simulink model "UkfSensorlessFOC"  (R2026b)
settings: Solver=FixedStepDiscrete  StopTime=experimentCfg.Duration  FixedStep=experimentCfg.Step
PostLoadFcn:
  | addpath(fullfile(fileparts(get_param(bdroot,'FileName')),'..','parameter'),fullfile(fileparts(get_param(bdroot,'FileName')),'..','build_process'));initialize_extension_foc(bdroot,'ukf');
model workspace (MAT data in the model file):
  bridgeCfg.Rs = 0.5
  bridgeCfg.Ld = 0.001
  bridgeCfg.Lq = 0.001
  bridgeCfg.Flux = 0.035
  bridgeCfg.PolePairs = 4
  bridgeCfg.J = 0.0005
  bridgeCfg.B = 0.0001
  bridgeCfg.Id0 = 0
  bridgeCfg.Iq0 = 0
  bridgeCfg.Speed0 = 0
  bridgeCfg.Position0 = 0.1
  bridgeCfg.Ts = 5e-06
  bridgeCfg.Vdc = 48
  bridgeCfg.DiodeVf = 0.7
  bridgeCfg.DiodeRon = 0.01
  bridgeCfg.MechanicalEnabled = 1
  bridgeCfg.CurrentTolerance = 1e-09
  bridgeCfg.VoltageTolerance = 1e-08
  bridgeCfg.MaxCurrent = 200
  bridgeCfg.MaxSpeed = 1000
  bridgeCfg.MaxAngleStep = 0.1
  bridgeCfg.State0 = [0; 0; 0; 0.1]
  bridgeCfg.Vector = [5e-06; 0.5; 0.001; 0.001; 0.035; 4; 0.0005; 0.0001; 48; 0.7; 0.01; 1; 1e-09; 1e-08; 200; 1000; 0.1]
  currentCfg.Ts = 5e-05
  currentCfg.BandwidthHz = 500
  currentCfg.Kpd = 3.14159265359
  currentCfg.Kpq = 3.14159265359
  currentCfg.Kid = 1570.79632679
  currentCfg.Kiq = 1570.79632679
  currentCfg.Kaw = 20000
  experimentCfg.UseTiming = 1
  experimentCfg.Step = 5e-06
  experimentCfg.Duration = 2.2
  extensionCfg.Kind = 'ukf'
  focCfg.Direction = 1
  focCfg.SpeedReference = 80
  focCfg.SpeedInitial = 0
  focCfg.CommandTime = 0.05
  focCfg.LoadTorque = 0.1
  focCfg.LoadTime = 0.9
  focCfg.Enable = 1
  focCfg.Reset = 0
  focCfg.ObserverEnable = 1
  focCfg.VoltageAlignmentEnable = 1
  focCfg.AlignmentVoltageGain = 0.5
  focCfg.FrameCorrectionTolerance = 1e-10
  fwCfg.BusTimes = 0
  fwCfg.BusValues = 48
  handoverCfg.Ts = 5e-05
  handoverCfg.MinOmega = 100
  handoverCfg.MaxSpeedGap = 80
  handoverCfg.MaxPhaseGap = 0.9
  handoverCfg.MaxResidual = 1.5
  handoverCfg.CaptureTime = 0.01
  handoverCfg.BlendTime = 0.1
  handoverCfg.LossTime = 0.001
  handoverCfg.MaxPhaseInnovation = 0.15
  handoverCfg.AllowFlying = 0
  handoverCfg.Samples = [200; 2000; 20]
  handoverCfg.Vector = [5e-05; 100; 80; 0.9; 1.5; 200; 2000; 20; 0.15; 0]
  handoverCfg.State0 = [0; 0; 0; 0; 0; 0; 0; 0; 0]
  inverterCfg.Vdc = 48
  inverterCfg.MinDuty = 0.02
  inverterCfg.PwmTs = 5e-05
  inverterCfg.LinearLimit = 26.6043004043
  motionCfg.SpeedLimit = 120
  motionCfg.AccelerationLimit = 200
  normalizedInverterCfg.Vdc = 1
  normalizedInverterCfg.MinDuty = 0.02
  normalizedInverterCfg.PwmTs = 5e-05
  normalizedInverterCfg.LinearLimit = 0.554256258422
  observerCfg.Model.Ts = 5e-05
  observerCfg.Model.Rs = 0.5
  observerCfg.Model.L = 0.001
  observerCfg.Model.Flux = 0.035
  observerCfg.Model.PolePairs = 4
  observerCfg.InitialOmega = 0
  observerCfg.InitialAngle = 0
  observerCfg.InitialStd = [1; 1; 500; 0.5]
  observerCfg.ProcessNoiseDensity = [2; 2; 2000; 1e-05]
  observerCfg.MeasurementStd = [0.002; 0.002]
  observerCfg.QualificationTime = 0.02
  observerCfg.MinOmega = 30
  observerCfg.MinEmf = 1
  observerCfg.MaxNIS = 25
  observerCfg.MaxThetaStd = 0.12
  observerCfg.MaxOmegaStd = 100
  observerCfg.AngleRateTimeConstant = 0.002
  observerCfg.MaxRateMismatch = 60
  observerCfg.MaxOmega = 2000
  observerCfg.MaxInputCurrent = 100
  observerCfg.MaxInputVoltage = 1000
  observerCfg.InitialVariance = [1; 1; 250000; 0.25]
  observerCfg.ProcessVariance = [0.0001; 0.0001; 0.1; 5e-10]
  observerCfg.MeasurementVariance = [4e-06; 4e-06]
  observerCfg.QualificationSamples = 400
  observerCfg.AngleRateAlpha = 0.0243902439024
  observerCfg.Settings = [5e-05; 0.5; 0.001; 0.035; 0; 0; 1; 1; 250000; 0.25; 0.0001; 0.0001; 0.1; 5e-10; 4e-06; 4e-06; 400; 30; 1; 25; 0.12; 100; 0.0243902439024; 60; 2000; 100; 1000]
  observerCfg.Alpha = 1
  observerCfg.Beta = 2
  observerCfg.Kappa = 0
  observerCfg.StateScales = [1; 1; 100; 1]
  observerCfg.InitialJitter = 1e-12
  observerCfg.MaximumJitter = 1e-08
  observerCfg.MaximumJitterAttempts = 5
  observerCfg.MinimumAngleResultant = 1e-06
  observerCfg.MaximumSigmaAngleDeviation = 1.56979632679
  observerCfg.UnscentedSettings = [5e-05; 0.5; 0.001; 0.035; 0; 0; 1; 1; 250000; 0.25; 0.0001; 0.0001; 0.1; 5e-10; 4e-06; 4e-06; 400; 30; 1; 25; 0.12; 100; 0.0243902439024; 60; 2000; 100; 1000; 1; 2; 0; 1; 1; 100; 1; 1e-12; 1e-08; 5; 1e-06; 1.56979632679]
  observerCfg.SigmaScale = 4
  observerCfg.MeanWeights = [0; 0.125; 0.125; 0.125; 0.125; 0.125; 0.125; 0.125; 0.125]
  observerCfg.CovarianceWeights = [2; 0.125; 0.125; 0.125; 0.125; 0.125; 0.125; 0.125; 0.125]
  pmsmCfg.Rs = 0.5
  pmsmCfg.Ld = 0.001
  pmsmCfg.Lq = 0.001
  pmsmCfg.Flux = 0.035
  pmsmCfg.PolePairs = 4
  pmsmCfg.J = 0.0005
  pmsmCfg.B = 0.0001
  pmsmCfg.Id0 = 0
  pmsmCfg.Iq0 = 0
  pmsmCfg.Speed0 = 0
  pmsmCfg.Position0 = 0.1
  refCfg.MtpaEnable = 0
  refCfg.FwEnable = 0
  refCfg.CurrentMax = 8
  refCfg.IdMin = -7
  refCfg.VoltageReserve = 0.95
  refCfg.FwVoltageMargin = 0.2
  refCfg.MinDuty = 0.02
  refCfg.FwTs = 0.001
  refCfg.FilterTau = 0.003
  refCfg.FwKi = 50
  refCfg.IdSlew = 200
  refCfg.TablePoints = 257
  refCfg.SpeedTs = 0.001
  refCfg.SpeedKp = 0.0179
  refCfg.SpeedKi = 0.2
  refCfg.SpeedKaw = 1000
  refCfg.IdTable = [0 0 0 0 0 0 0 0 0 0 0 0 0 0 0 0 0 0 0 0 0 0 0 0 0 0 0 0 0 0 0 0 0 0 0 0 0 0 0 0 0 0 0 0 0 0 0 0 0 0 0 0 0 0 0 0 0 0 0 0 0 0 0 0 0 0 0 0 0 0 0 0 0 0 0 0 0 0 0 0 0 0 0 0 0 0 0 0 0 0 0 0 0 0 0 0 0 0 0 0 0 0 0 0 0 0 0 0 0 0 0 0 0 0 0 0 0 0 0 0 0 0 0 0 0 0 0 0 0 0 0 0 0 0 0 0 0 0 0 0 0 0 0 0 0 0 0 0 0 0 0 0 0 0 0 0 0 0 0 0 0 0 0 0 0 0 0 0 0 0 0 0 0 0 0 0 0 0 0 0 0 0 0 0 0 0 0 0 0 0 0 0 0 0 0 0 0 0 0 0 0 0 0 0 0 0 0 0 0 0 0 0 0 0 0 0 0 0 0 0 0 0 0 0 0 0 0 0 0 0 0 0 0 0 0 0 0 0 0 0 0 0 0 0 0 0 0 0 0 0 0 0 0 0 0 0 0]
  refCfg.TorqueGrid = [0 0.0065625 0.013125 0.0196875 0.02625 0.0328125 0.039375 0.0459375 0.0525 0.0590625 0.065625 0.0721875 ... (257 elements, 1x257)]
  refCfg.MaxTorque = 1.68
  refCfg.Kt = 0.21
  refCfg.VoltageFactor = 0.526543445501
  refCfg.FilterAlpha = 0.75
  startGuardCfg.Enable = 1
  startGuardCfg.ObserveTime = 0.05
  startGuardCfg.ObserveTicks = 1000
  startGuardCfg.MaxStartVoltage = 0.25
  startupCfg.Ts = 5e-05
  startupCfg.Theta0 = 0
  startupCfg.AlignCurrent = 2
  startupCfg.StartupCurrent = 3
  startupCfg.FinalOmega = 250
  startupCfg.FlyingCaptureTime = 0.03
  startupCfg.PrealignTime = 0.06
  startupCfg.PrealignRampTime = 0.03
  startupCfg.AlignTime = 0.08
  startupCfg.AlignRampTime = 0.04
  startupCfg.OmegaRampTime = 0.35
  startupCfg.CurrentRampTime = 0.05
  startupCfg.MinCaptureOmega = 150
  startupCfg.MaxIFTime = 0.8
  startupCfg.Samples = [600 1200 600 1600 800 7000 1000 16000]
  startupCfg.Vector = [5e-05; 0; 2; 3; 250; 600; 1200; 600; 1600; 800; 7000; 1000; 16000; 150]
  startupCfg.State0 = [0; 0; 0; 0; 0]
  testStim.time = [0 5e-05 0.0001 0.00015 0.0002 0.00025 0.0003 0.00035 0.0004 0.00045 0.0005 0.00055 ... (44001 elements, 44001x1)]
  testStim.signals.values = [0 0 0 0 0 0 0 0 0 0 0 0 ... (308007 elements, 44001x7)]
  testStim.signals.dimensions = 7
  timingCfg.Ts = 5e-05
  timingCfg.FeedbackTicks = 0
  timingCfg.ActuationTicks = 1
libraries: ClarkePark x9, CurrentReference x2, CurrentControl x2, Inverter x2, SensorlessHandover x1, SensorlessStartup x1, UkfObserver x1, PMSMBridgeBusPlant x1, ControlTiming x1
settings Model: Creator=24322  LastModifiedBy=24322
settings DebuggingCC: AlgebraicLoopMsg=error

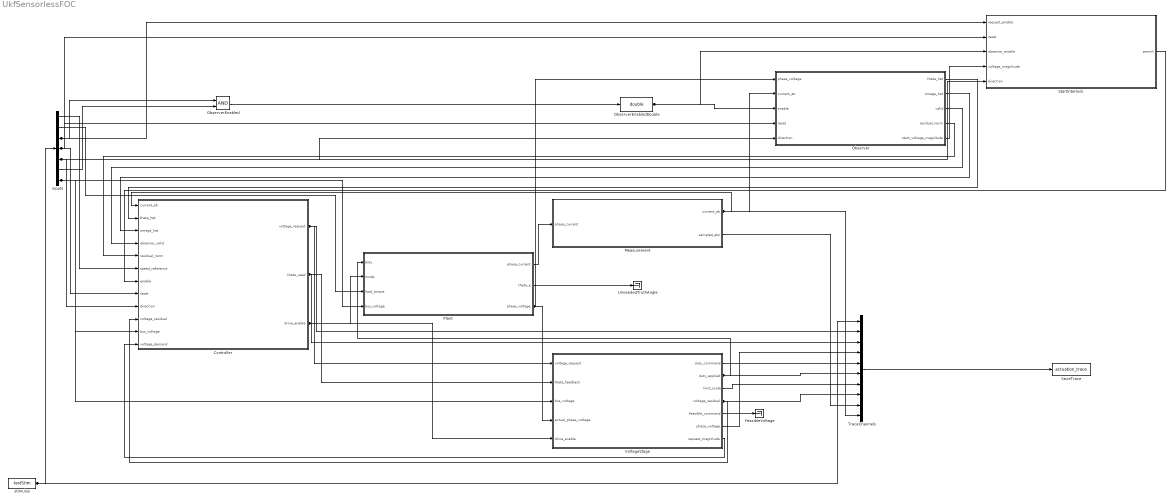
== system UkfSensorlessFOC ==
  Controller : Subsystem
  FeasibleVoltage : Terminator
  Measurement : Subsystem
  Observer : Subsystem
  ObserverEnabled : Logic  IconShape=distinctive  AllPortsSameDT=off  OutDataTypeStr=boolean
  ObserverEnabledDouble : DataTypeConversion  OutDataTypeStr=double  SaturateOnIntegerOverflow=off  RndMeth=Floor
  Plant : Subsystem
  SaveTrace : ToWorkspace  VariableName=actuation_trace  SaveFormat=Structure With Time  SampleTime=currentCfg.Ts
  StartInterlock : Subsystem
  TraceChannels : Mux  Inputs=10
  UnneededTruthAngle : Terminator
  VoltageStage : Subsystem  mask{inverterCfg=normalizedInverterCfg}
      mask prompts: inverterCfg "Normalized inverter configuration"
  inputs : Demux  Outputs=7
  stimulus : FromWorkspace  VariableName=testStim  SampleTime=currentCfg.Ts  Interpolate=off  OutputAfterFinalValue=Holding final value
  wires:
  inputs/7 -> Controller/11(bus_voltage), Plant/4(bus_voltage), VoltageStage/3(bus_voltage)
  inputs/5 -> Controller/9(direction), StartInterlock/5(direction), Observer/5(direction)
  inputs/4 -> Controller/8(reset), StartInterlock/2(reset), Observer/4(reset)
  inputs/3 -> ObserverEnabled/1, StartInterlock/1(request_enable)
  inputs/1 -> Controller/6(speed_reference)
  ObserverEnabled/1 -> ObserverEnabledDouble/1
  VoltageStage/7(request_magnitude) -> Controller/12(voltage_demand)
  VoltageStage/4(voltage_residual) -> TraceChannels/8, Controller/10(voltage_residual)
  Controller/3(drive_enable) -> Plant/2(mode), VoltageStage/5(drive_enable)
  Plant/3(phase_voltage) -> VoltageStage/4(actual_phase_voltage), Observer/1(phase_voltage)
  Controller/2(theta_used) -> TraceChannels/3, VoltageStage/2(theta_feedback)
  Controller/1(voltage_request) -> TraceChannels/2, VoltageStage/1(voltage_request)
  Measurement/1(current_ab) -> TraceChannels/10, Controller/1(current_ab), Observer/2(current_ab)
  ObserverEnabledDouble/1 -> StartInterlock/3(observer_enable), Observer/3(enable)
  StartInterlock/1(permit) -> Controller/7(enable)
  VoltageStage/2(duty_applied) -> Plant/1(duty), TraceChannels/6
  Plant/1(phase_current) -> Measurement/1(phase_current)
  Plant/2(theta_e) -> UnneededTruthAngle/1
  inputs/2 -> Plant/3(load_torque)
  Measurement/2(sampled_abc) -> TraceChannels/9
  Observer/5(start_voltage_magnitude) -> StartInterlock/4(voltage_magnitude)
  Observer/1(theta_hat) -> Controller/2(theta_hat)
  Observer/2(omega_hat) -> Controller/3(omega_hat)
  Observer/3(valid) -> Controller/4(observer_valid)
  Observer/4(residual_norm) -> Controller/5(residual_norm)
  TraceChannels/1 -> SaveTrace/1
  inputs/6 -> ObserverEnabled/2
  VoltageStage/3(limit_scale) -> TraceChannels/7
  VoltageStage/1(duty_command) -> TraceChannels/5
  VoltageStage/6(phase_voltage) -> TraceChannels/4
  VoltageStage/5(feasible_command) -> FeasibleVoltage/1
  stimulus/1 -> TraceChannels/1, inputs/1

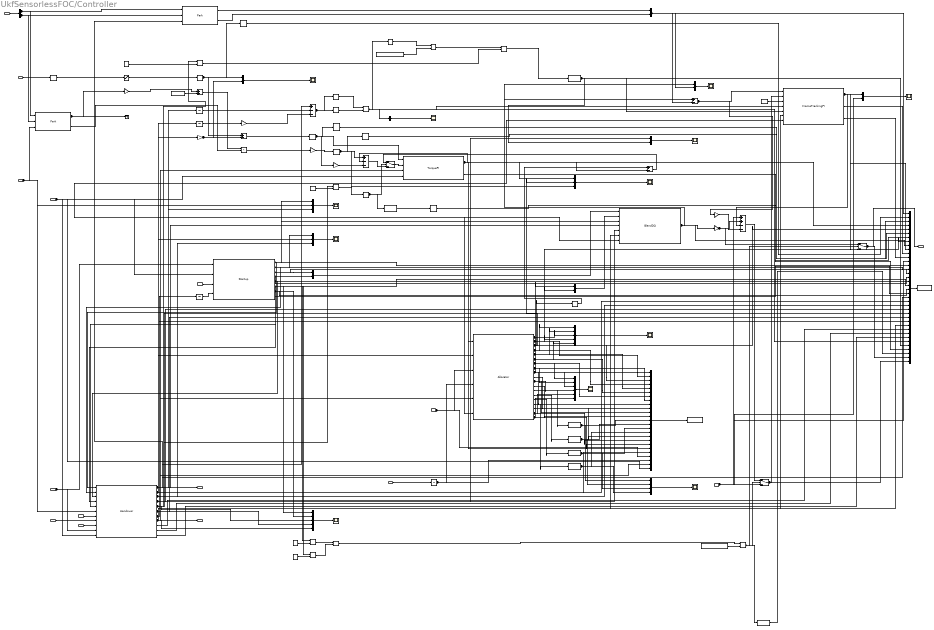
== system UkfSensorlessFOC/Controller ==
  current_ab : Inport
  theta_hat : Inport  Port=2
  omega_hat : Inport  Port=3
  observer_valid : Inport  Port=4
  residual_norm : Inport  Port=5
  speed_reference : Inport  Port=6
  enable : Inport  Port=7
  reset : Inport  Port=8
  direction : Inport  Port=9
  voltage_residual : Inport  Port=10
  bus_voltage : Inport  Port=11
  voltage_demand : Inport  Port=12
  AcquiredDelay : UnitDelay  SampleTime=currentCfg.Ts
  AlignMode : Constant  Value=3
  AlignmentIntegralCancellation : Gain  Gain=diag([currentCfg.Kid,currentCfg.Kiq])/max(currentCfg.Kaw,eps)  Multiplication=Matrix(K*u)
  AlignmentResidual : Sum  Inputs=++--
  AlignmentStage : Logic  Operator=OR  IconShape=distinctive  AllPortsSameDT=off  OutDataTypeStr=boolean
  AlignmentVoltage : Gain  Gain=focCfg.AlignmentVoltageGain
  AllocatedTorqueSample : ZeroOrderHold  SampleTime=refCfg.SpeedTs
  AllocationChannels : Mux  Inputs=25
  AllocationFlagsScope : Scope
  AllocationFlagsScopeChannels : Mux
  AllocationVoltageScope : Scope
  AllocationVoltageScopeChannels : Mux  Inputs=6
  AngleScope : Scope
  AngleScope_mux : Mux  Inputs=3
  AutoDouble : DataTypeConversion  OutDataTypeStr=double  SaturateOnIntegerOverflow=off  RndMeth=Floor
  AutoMode : Constant  Value=4
  AutoSample : ZeroOrderHold  SampleTime=refCfg.SpeedTs
  BlendMode : Constant  Value=3
  ClosedCurrent : Mux  Inputs=2
  ControlCurrent : Mux  Inputs=2
  ControlPark : ClarkePark/Park  SystemSampleTime=-1  VariantActivationTime=update diagram  EmptyChoice=off  PassThrough=off  PassThroughVariantControl=(default)  EmptyChoiceVariantControl=(default)  AllowFlexibleInterface=on  Latency=0  AutoFrameSizeCalculation=off
  CorrectionTolerance : Constant  Value=focCfg.FrameCorrectionTolerance
  CurrentAllocationScope : Scope
  CurrentAllocationScopeChannels : Mux  Inputs=5
  CurrentAllocator : CurrentReference/Allocator  SystemSampleTime=-1  VariantActivationTime=update diagram  EmptyChoice=off  PassThrough=off  PassThroughVariantControl=(default)  EmptyChoiceVariantControl=(default)  AllowFlexibleInterface=on  Latency=0  AutoFrameSizeCalculation=off
  CurrentChannels : Demux  Outputs=2
  CurrentError : Sum  Inputs=+-
  CurrentLimitFlagDouble : DataTypeConversion  OutDataTypeStr=double  SaturateOnIntegerOverflow=off  RndMeth=Floor
  CurrentPI : CurrentControl/FrameTrackingPI  currentCfg=currentCfg
  CurrentScope : Scope
  CurrentScope_mux : Mux  Inputs=2
  EstimatedActiveFlux : Sum
  EstimatedDCurrent : Terminator
  EstimatedFlux : Constant  Value=pmsmCfg.Flux
  EstimatedRotorPark : ClarkePark/Park  SystemSampleTime=-1  VariantActivationTime=update diagram  EmptyChoice=off  PassThrough=off  PassThroughVariantControl=(default)  EmptyChoiceVariantControl=(default)  AllowFlexibleInterface=on  Latency=0  AutoFrameSizeCalculation=off
  EstimatedSaliency : Gain  Gain=pmsmCfg.Ld-pmsmCfg.Lq
  EstimatedTorque : Gain  Gain=1.5*pmsmCfg.PolePairs
  EstimatedTorqueProduct : Product  Inputs=**
  EstimatedTorqueSample : ZeroOrderHold  SampleTime=refCfg.SpeedTs
  ExtraAngle : Trigonometry  Operator=atan2
  ExtraAngleScope : Scope
  ExtraAngleScope_mux : Mux  Inputs=1
  ExtraCos : Trigonometry  Operator=cos
  ExtraMagnitude : Abs  SaturateOnIntegerOverflow=off
  ExtraSin : Trigonometry
  FeasibleFlagDouble : DataTypeConversion  OutDataTypeStr=double  SaturateOnIntegerOverflow=off  RndMeth=Floor
  FrameSpeedScope : Scope
  FrameSpeedScope_mux : Mux  Inputs=3
  Handover : SensorlessHandover/Handover  handoverCfg=handoverCfg
  HasCorrection : RelationalOperator  Operator=>  OutDataTypeStr=boolean  RndMeth=Simplest  InputSameDT=off
  IntegralTrackingCancellation : Gain  Gain=refCfg.SpeedKi/refCfg.SpeedKaw
  IsAlign : RelationalOperator  Operator===  OutDataTypeStr=boolean  RndMeth=Simplest  InputSameDT=off
  IsAuto : RelationalOperator  Operator===  OutDataTypeStr=boolean  RndMeth=Simplest  InputSameDT=off
  IsBlending : RelationalOperator  Operator===  OutDataTypeStr=boolean  RndMeth=Simplest  InputSameDT=off
  IsPrealign : RelationalOperator  Operator===  OutDataTypeStr=boolean  RndMeth=Simplest  InputSameDT=off
  LogRate_auto_sampled : RateTransition  Integrity=off  Deterministic=off  OutPortSampleTime=currentCfg.Ts
  LogRate_speed_error : RateTransition  Integrity=off  Deterministic=off  OutPortSampleTime=currentCfg.Ts
  LogRate_speed_reference : RateTransition  Integrity=off  Deterministic=off  OutPortSampleTime=currentCfg.Ts
  LogRate_torque_estimated : RateTransition  Integrity=off  Deterministic=off  OutPortSampleTime=currentCfg.Ts
  MechanicalEstimate : Gain  Gain=1/pmsmCfg.PolePairs
  NominalAngleStep : Gain  Gain=currentCfg.Ts
  NormalTorqueResidual : Sum  Inputs=+-
  PIResidualUsed : Switch  Criteria=u2 ~= 0  SaturateOnIntegerOverflow=off  InputSameDT=off
  PrealignMode : Constant  Value=2
  PreviousAngle : UnitDelay  SampleTime=currentCfg.Ts
  PreviousOmega : UnitDelay  SampleTime=currentCfg.Ts
  RawExtraAngle : Sum  Inputs=+--
  ReferenceBlend : ClarkePark/BlendDQ  SystemSampleTime=-1  VariantActivationTime=update diagram  EmptyChoice=off  PassThrough=off  PassThroughVariantControl=(default)  EmptyChoiceVariantControl=(default)  AllowFlexibleInterface=on  Latency=0  AutoFrameSizeCalculation=off
  SaveAllocation : ToWorkspace  VariableName=allocation_trace  SaveFormat=Structure With Time  SampleTime=currentCfg.Ts
  SaveTrace : ToWorkspace  VariableName=controller_trace  SaveFormat=Structure With Time  SampleTime=currentCfg.Ts
  SpeedError : Sum  Inputs=+-
  SpeedErrorSample : ZeroOrderHold  SampleTime=refCfg.SpeedTs
  SpeedLoopScope : Scope
  SpeedLoopScope_mux : Mux  Inputs=2
  SpeedPI : CurrentReference/TorquePI  SystemSampleTime=-1  VariantActivationTime=update diagram  EmptyChoice=off  PassThrough=off  PassThroughVariantControl=(default)  EmptyChoiceVariantControl=(default)  AllowFlexibleInterface=on  Latency=0  AutoFrameSizeCalculation=off
  SpeedReferenceLimit : Saturate  UpperLimit=motionCfg.SpeedLimit  LowerLimit=-motionCfg.SpeedLimit
  SpeedReferenceSample : ZeroOrderHold  SampleTime=refCfg.SpeedTs
  SpeedReferenceSlew : RateLimiter  RisingSlewLimit=motionCfg.AccelerationLimit  FallingSlewLimit=-motionCfg.AccelerationLimit  SampleTimeMode=inherited
  Startup : SensorlessStartup/Startup  startupCfg=startupCfg
  StartupCurrent : Mux  Inputs=2
  StateScope : Scope
  StateScope_mux : Mux  Inputs=5
  TorqueLoopScope : Scope
  TorqueLoopScope_mux : Mux  Inputs=3
  TorqueResidual : Switch  Criteria=u2 ~= 0  SaturateOnIntegerOverflow=off  InputSameDT=off
  TraceChannels : Mux  Inputs=38
  TrackDouble : DataTypeConversion  OutDataTypeStr=double  SaturateOnIntegerOverflow=off  RndMeth=Floor
  TrackLogic : Logic  Operator=OR  IconShape=distinctive  AllPortsSameDT=off  OutDataTypeStr=boolean
  TrackingTorqueResidual : Sum  Inputs=+--
  TransitionScope : Scope
  TransitionScope_mux : Mux  Inputs=2
  UseVoltageAlignment : Logic  IconShape=distinctive  AllPortsSameDT=off  OutDataTypeStr=boolean
  VoltageAlignDouble : DataTypeConversion  OutDataTypeStr=double  SaturateOnIntegerOverflow=off  RndMeth=Floor
  VoltageAlignmentEnabled : Constant  Value=focCfg.VoltageAlignmentEnable
  VoltageDemandPrevious : UnitDelay  SampleTime=currentCfg.Ts
  VoltageLimitFlagDouble : DataTypeConversion  OutDataTypeStr=double  SaturateOnIntegerOverflow=off  RndMeth=Floor
  VoltageScope : Scope
  VoltageScope_mux : Mux  Inputs=2
  VoltageSelected : Switch  Criteria=u2 ~= 0  SaturateOnIntegerOverflow=off  InputSameDT=off
  WeakeningFlagDouble : DataTypeConversion  OutDataTypeStr=double  SaturateOnIntegerOverflow=off  RndMeth=Floor
  ZeroVector : Constant  Value=[0;0]
  voltage_request : Outport
  theta_used : Outport  Port=2
  drive_enable : Outport  Port=3
  wires:
  current_ab/1 -> CurrentChannels/1
  CurrentAllocator/17 -> AllocationChannels/17
  WeakeningFlagDouble/1 -> AllocationChannels/16, AllocationFlagsScopeChannels/4
  FeasibleFlagDouble/1 -> AllocationChannels/15, AllocationFlagsScopeChannels/3
  VoltageLimitFlagDouble/1 -> AllocationChannels/14, AllocationFlagsScopeChannels/2
  CurrentLimitFlagDouble/1 -> AllocationChannels/13, AllocationFlagsScopeChannels/1
  CurrentAllocator/12 -> AllocationChannels/12
  CurrentAllocator/10 -> AllocationChannels/10
  CurrentAllocator/15 -> FeasibleFlagDouble/1
  CurrentAllocator/14 -> VoltageLimitFlagDouble/1
  CurrentAllocator/13 -> CurrentLimitFlagDouble/1
  AllocationFlagsScopeChannels/1 -> AllocationFlagsScope/1
  AllocationChannels/1 -> SaveAllocation/1
  CurrentAllocator/16 -> WeakeningFlagDouble/1
  AllocationVoltageScopeChannels/1 -> AllocationVoltageScope/1
  CurrentAllocationScopeChannels/1 -> CurrentAllocationScope/1
  CurrentAllocator/19 -> AllocationVoltageScopeChannels/6, AllocationChannels/19
  CurrentAllocator/18 -> AllocationVoltageScopeChannels/5, AllocationChannels/18
  CurrentAllocator/11 -> AllocationVoltageScopeChannels/4, AllocationChannels/11
  CurrentAllocator/9 -> AllocationVoltageScopeChannels/3, AllocationChannels/9
  CurrentAllocator/8 -> AllocationVoltageScopeChannels/2, AllocationChannels/8
  CurrentAllocator/7 -> AllocationVoltageScopeChannels/1, AllocationChannels/7
  CurrentAllocator/6 -> CurrentAllocationScopeChannels/5, AllocationChannels/6
  CurrentAllocator/5 -> CurrentAllocationScopeChannels/2, AllocationChannels/5
  CurrentAllocator/4 -> CurrentAllocationScopeChannels/1, AllocationChannels/4
  EstimatedTorque/1 -> EstimatedTorqueSample/1
  CurrentAllocator/3 -> TraceChannels/5, AllocationChannels/3, AllocatedTorqueSample/1, TorqueLoopScope_mux/2
  CurrentAllocator/2 -> TraceChannels/8, ClosedCurrent/2, CurrentAllocationScopeChannels/4, AllocationChannels/2
  EstimatedTorqueProduct/1 -> EstimatedTorque/1
  EstimatedRotorPark/2 -> EstimatedTorqueProduct/2
  EstimatedActiveFlux/1 -> EstimatedTorqueProduct/1
  EstimatedFlux/1 -> EstimatedActiveFlux/2
  EstimatedSaliency/1 -> EstimatedActiveFlux/1
  CurrentAllocator/1 -> ClosedCurrent/1, CurrentAllocationScopeChannels/3, AllocationChannels/1
  VoltageDemandPrevious/1 -> CurrentAllocator/4, AllocationChannels/23
  voltage_demand/1 -> VoltageDemandPrevious/1
  bus_voltage/1 -> CurrentAllocator/3, AllocationChannels/22
  VoltageScope_mux/1 -> VoltageScope/1
  TorqueLoopScope_mux/1 -> TorqueLoopScope/1
  SpeedLoopScope_mux/1 -> SpeedLoopScope/1
  StateScope_mux/1 -> StateScope/1
  ExtraAngleScope_mux/1 -> ExtraAngleScope/1
  TransitionScope_mux/1 -> TransitionScope/1
  FrameSpeedScope_mux/1 -> FrameSpeedScope/1
  AngleScope_mux/1 -> AngleScope/1
  CurrentScope_mux/1 -> CurrentScope/1
  AutoDouble/1 -> LogRate_auto_sampled/1
  Handover/11 -> TraceChannels/32
  Handover/10 -> TraceChannels/31
  Handover/9 -> TraceChannels/30
  Handover/6 -> TraceChannels/27, StateScope_mux/4
  Handover/3 -> TraceChannels/24, FrameSpeedScope_mux/3
  Startup/8 -> TraceChannels/21
  CurrentPI/3 -> TraceChannels/12
  CurrentPI/2 -> TraceChannels/11
  SpeedPI/2 -> TraceChannels/7
  TraceChannels/1 -> SaveTrace/1
  TrackLogic/1 -> TrackDouble/1
  IsBlending/1 -> TrackLogic/2
  HasCorrection/1 -> TrackLogic/1
  BlendMode/1 -> IsBlending/2
  CorrectionTolerance/1 -> HasCorrection/2
  ExtraMagnitude/1 -> HasCorrection/1
  ExtraCos/1 -> ExtraAngle/2
  ExtraSin/1 -> ExtraAngle/1
  RawExtraAngle/1 -> ExtraSin/1, ExtraCos/1
  NominalAngleStep/1 -> RawExtraAngle/3
  PreviousAngle/1 -> RawExtraAngle/2
  PreviousOmega/1 -> NominalAngleStep/1
  Handover/2 -> PreviousOmega/1, AllocationChannels/21, TraceChannels/23, FrameSpeedScope_mux/2, MechanicalEstimate/1, CurrentAllocator/2
  CurrentPI/1 -> VoltageScope_mux/1, VoltageSelected/3, AlignmentResidual/3, TraceChannels/10
  TrackDouble/1 -> TraceChannels/34, TransitionScope_mux/2, CurrentPI/5
  ExtraAngle/1 -> ExtraAngleScope_mux/1, ExtraMagnitude/1, TraceChannels/33, CurrentPI/4
  ZeroVector/1 -> CurrentPI/3
  voltage_residual/1 -> VoltageScope_mux/2, PIResidualUsed/3, AlignmentResidual/1, TraceChannels/13
  CurrentError/1 -> AlignmentIntegralCancellation/1, CurrentPI/1
  ControlCurrent/1 -> CurrentError/2, TraceChannels/1, CurrentScope_mux/2
  ReferenceBlend/1 -> CurrentScope_mux/1, TraceChannels/9, AlignmentVoltage/1, CurrentError/1
  Handover/4 -> TransitionScope_mux/1, TraceChannels/25, ReferenceBlend/5
  ClosedCurrent/1 -> ReferenceBlend/2
  StartupCurrent/1 -> ReferenceBlend/1
  Startup/4 -> StartupCurrent/2, TraceChannels/17
  Startup/3 -> StartupCurrent/1, TraceChannels/16
  TrackingTorqueResidual/1 -> TorqueResidual/3
  NormalTorqueResidual/1 -> TorqueResidual/1
  AutoSample/1 -> AutoDouble/1, TorqueResidual/2
  IsAuto/1 -> AutoSample/1
  AutoMode/1 -> IsAuto/2
  Handover/5 -> IsAuto/1, IsBlending/1, TraceChannels/26, StateScope_mux/3
  IntegralTrackingCancellation/1 -> TrackingTorqueResidual/3
  EstimatedTorqueSample/1 -> LogRate_torque_estimated/1, TrackingTorqueResidual/1, TorqueLoopScope_mux/3
  AllocatedTorqueSample/1 -> NormalTorqueResidual/1
  SpeedPI/1 -> NormalTorqueResidual/2, TrackingTorqueResidual/2, TraceChannels/4, CurrentAllocator/1, TorqueLoopScope_mux/1, AllocationChannels/20
  Handover/8 -> TraceChannels/29, StateScope_mux/5, CurrentAllocator/5, drive_enable/1, AllocationChannels/24, CurrentPI/6, SpeedPI/3, ReferenceBlend/6
  TorqueResidual/1 -> SpeedPI/2
  SpeedErrorSample/1 -> LogRate_speed_error/1, IntegralTrackingCancellation/1, SpeedPI/1
  SpeedError/1 -> SpeedErrorSample/1
  MechanicalEstimate/1 -> SpeedError/2, SpeedLoopScope_mux/2
  SpeedReferenceSlew/1 -> LogRate_speed_reference/1, SpeedLoopScope_mux/1, SpeedError/1
  SpeedReferenceLimit/1 -> SpeedReferenceSlew/1
  SpeedReferenceSample/1 -> SpeedReferenceLimit/1
  speed_reference/1 -> SpeedReferenceSample/1
  residual_norm/1 -> Handover/9
  observer_valid/1 -> Handover/8
  omega_hat/1 -> Handover/7
  Startup/7 -> StateScope_mux/2, Handover/5, TraceChannels/20
  Startup/6 -> TraceChannels/19, IsAlign/1, IsPrealign/1, Handover/4, StateScope_mux/1
  Startup/5 -> Handover/3, TraceChannels/18
  Startup/2 -> FrameSpeedScope_mux/1, Handover/2, TraceChannels/15
  Startup/1 -> AngleScope_mux/1, TraceChannels/14, ReferenceBlend/3, Handover/1
  Handover/7 -> TraceChannels/28, AcquiredDelay/1
  AcquiredDelay/1 -> Startup/4
  direction/1 -> Startup/3
  reset/1 -> Handover/11, CurrentPI/7, ReferenceBlend/7, AllocationChannels/25, CurrentAllocator/6, Startup/2, SpeedPI/4
  enable/1 -> Startup/1, Handover/10
  EstimatedRotorPark/1 -> EstimatedDCurrent/1, EstimatedSaliency/1
  theta_hat/1 -> AngleScope_mux/2, Handover/6, EstimatedRotorPark/3
  ControlPark/2 -> ControlCurrent/2
  ControlPark/1 -> ControlCurrent/1
  Handover/1 -> ReferenceBlend/4, theta_used/1, RawExtraAngle/1, TraceChannels/22, PreviousAngle/1, AngleScope_mux/3, ControlPark/3
  CurrentChannels/2 -> ControlPark/2, EstimatedRotorPark/2
  CurrentChannels/1 -> ControlPark/1, EstimatedRotorPark/1
  PrealignMode/1 -> IsPrealign/2
  AlignMode/1 -> IsAlign/2
  IsPrealign/1 -> AlignmentStage/1
  IsAlign/1 -> AlignmentStage/2
  AlignmentStage/1 -> UseVoltageAlignment/1
  VoltageAlignmentEnabled/1 -> UseVoltageAlignment/2
  UseVoltageAlignment/1 -> VoltageSelected/2, PIResidualUsed/2, VoltageAlignDouble/1
  AlignmentVoltage/1 -> VoltageSelected/1, AlignmentResidual/2
  AlignmentIntegralCancellation/1 -> AlignmentResidual/4
  AlignmentResidual/1 -> PIResidualUsed/1
  PIResidualUsed/1 -> TraceChannels/38, CurrentPI/2
  VoltageSelected/1 -> TraceChannels/37, voltage_request/1
  LogRate_speed_reference/1 -> TraceChannels/2
  LogRate_speed_error/1 -> TraceChannels/3
  LogRate_torque_estimated/1 -> TraceChannels/6
  LogRate_auto_sampled/1 -> TraceChannels/35
  VoltageAlignDouble/1 -> TraceChannels/36

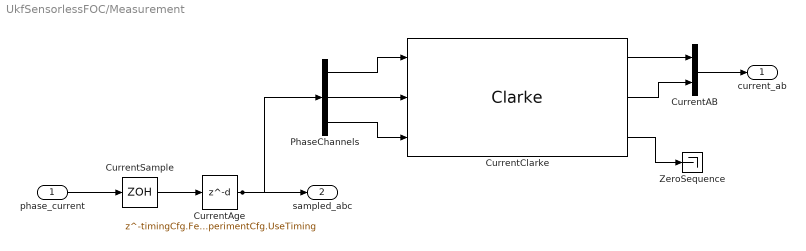
== system UkfSensorlessFOC/Measurement ==
  phase_current : Inport
  CurrentAB : Mux  Inputs=2
  CurrentAge : Delay  DelayLength=timingCfg.FeedbackTicks*experimentCfg.UseTiming  InitialCondition=0  SampleTime=timingCfg.Ts
  CurrentClarke : ClarkePark/Clarke  SystemSampleTime=-1  VariantActivationTime=update diagram  EmptyChoice=off  PassThrough=off  PassThroughVariantControl=(default)  EmptyChoiceVariantControl=(default)  AllowFlexibleInterface=on  Latency=0  AutoFrameSizeCalculation=off
  CurrentSample : ZeroOrderHold  SampleTime=timingCfg.Ts
  PhaseChannels : Demux  Outputs=3
  ZeroSequence : Terminator
  current_ab : Outport
  sampled_abc : Outport  Port=2
  wires:
  phase_current/1 -> CurrentSample/1
  CurrentSample/1 -> CurrentAge/1
  CurrentAge/1 -> sampled_abc/1, PhaseChannels/1
  CurrentClarke/1 -> CurrentAB/1
  CurrentClarke/2 -> CurrentAB/2
  CurrentClarke/3 -> ZeroSequence/1
  CurrentAB/1 -> current_ab/1
  PhaseChannels/1 -> CurrentClarke/1
  PhaseChannels/2 -> CurrentClarke/2
  PhaseChannels/3 -> CurrentClarke/3

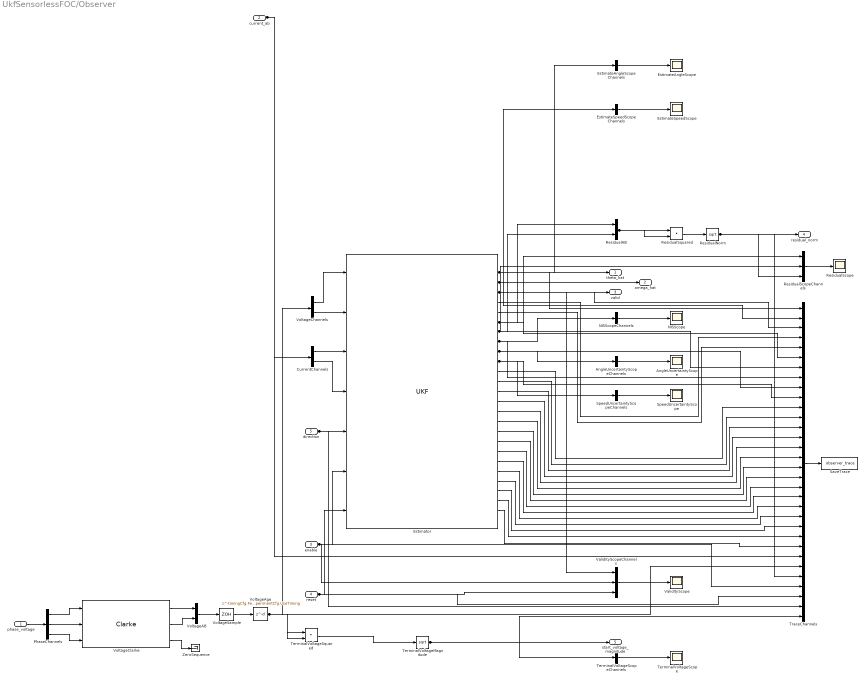
== system UkfSensorlessFOC/Observer ==
  phase_voltage : Inport
  current_ab : Inport  Port=2
  enable : Inport  Port=3
  reset : Inport  Port=4
  direction : Inport  Port=5
  AngleUncertaintyScope : Scope
  AngleUncertaintyScopeChannels : Mux  Inputs=1
  CurrentChannels : Demux  Outputs=2
  EstimateAngleScope : Scope
  EstimateAngleScopeChannels : Mux  Inputs=1
  EstimateSpeedScope : Scope
  EstimateSpeedScopeChannels : Mux  Inputs=1
  Estimator : UkfObserver/UKF  cfg=observerCfg
  NISScope : Scope
  NISScopeChannels : Mux  Inputs=1
  PhaseChannels : Demux  Outputs=3
  ResidualAB : Mux  Inputs=2
  ResidualNorm : Sqrt
  ResidualScope : Scope
  ResidualScopeChannels : Mux  Inputs=3
  ResidualSquared : DotProduct  OutDataTypeStr=Inherit: Inherit via internal rule
  SaveTrace : ToWorkspace  VariableName=observer_trace  SaveFormat=Structure With Time  SampleTime=currentCfg.Ts
  SpeedUncertaintyScope : Scope
  SpeedUncertaintyScopeChannels : Mux  Inputs=1
  TerminalVoltageMagnitude : Sqrt
  TerminalVoltageScope : Scope
  TerminalVoltageScopeChannels : Mux  Inputs=1
  TerminalVoltageSquared : DotProduct  OutDataTypeStr=Inherit: Inherit via internal rule
  TraceChannels : Mux  Inputs=32
  ValidityScope : Scope
  ValidityScopeChannels : Mux  Inputs=3
  VoltageAB : Mux  Inputs=2
  VoltageAge : Delay  DelayLength=timingCfg.FeedbackTicks*experimentCfg.UseTiming  InitialCondition=0  SampleTime=timingCfg.Ts
  VoltageChannels : Demux  Outputs=2
  VoltageClarke : ClarkePark/Clarke  SystemSampleTime=-1  VariantActivationTime=update diagram  EmptyChoice=off  PassThrough=off  PassThroughVariantControl=(default)  EmptyChoiceVariantControl=(default)  AllowFlexibleInterface=on  Latency=0  AutoFrameSizeCalculation=off
  VoltageSample : ZeroOrderHold  SampleTime=timingCfg.Ts
  ZeroSequence : Terminator
  theta_hat : Outport
  omega_hat : Outport  Port=2
  valid : Outport  Port=3
  residual_norm : Outport  Port=4
  start_voltage_magnitude : Outport  Port=5
  wires:
  phase_voltage/1 -> PhaseChannels/1
  current_ab/1 -> CurrentChannels/1, TraceChannels/26
  VoltageClarke/1 -> VoltageAB/1
  VoltageClarke/2 -> VoltageAB/2
  VoltageClarke/3 -> ZeroSequence/1
  VoltageAB/1 -> VoltageSample/1
  VoltageSample/1 -> VoltageAge/1
  VoltageAge/1 -> TerminalVoltageSquared/2, TerminalVoltageSquared/1, TraceChannels/27, VoltageChannels/1
  VoltageChannels/1 -> Estimator/1
  VoltageChannels/2 -> Estimator/2
  CurrentChannels/1 -> Estimator/3
  CurrentChannels/2 -> Estimator/4
  direction/1 -> TraceChannels/31, Estimator/5
  enable/1 -> TraceChannels/29, Estimator/6, ValidityScopeChannels/2
  reset/1 -> ValidityScopeChannels/3, Estimator/7, TraceChannels/30
  Estimator/1 -> EstimateAngleScopeChannels/1, TraceChannels/1, theta_hat/1
  Estimator/2 -> EstimateSpeedScopeChannels/1, TraceChannels/2, omega_hat/1
  Estimator/3 -> ValidityScopeChannels/1, TraceChannels/3, valid/1
  ResidualAB/1 -> ResidualSquared/2, ResidualSquared/1
  ResidualSquared/1 -> ResidualNorm/1
  ResidualNorm/1 -> ResidualScopeChannels/3, residual_norm/1, TraceChannels/28
  TerminalVoltageSquared/1 -> TerminalVoltageMagnitude/1
  TerminalVoltageMagnitude/1 -> TerminalVoltageScopeChannels/1, start_voltage_magnitude/1, TraceChannels/32
  PhaseChannels/1 -> VoltageClarke/1
  PhaseChannels/2 -> VoltageClarke/2
  PhaseChannels/3 -> VoltageClarke/3
  Estimator/6 -> ResidualScopeChannels/1, ResidualAB/1, TraceChannels/6
  Estimator/7 -> ResidualScopeChannels/2, TraceChannels/7, ResidualAB/2
  TraceChannels/1 -> SaveTrace/1
  Estimator/4 -> TraceChannels/4
  Estimator/5 -> TraceChannels/5
  Estimator/8 -> NISScopeChannels/1, TraceChannels/8
  Estimator/9 -> AngleUncertaintyScopeChannels/1, TraceChannels/9
  Estimator/10 -> SpeedUncertaintyScopeChannels/1, TraceChannels/10
  Estimator/11 -> TraceChannels/11
  Estimator/12 -> TraceChannels/12
  Estimator/13 -> TraceChannels/13
  Estimator/14 -> TraceChannels/14
  Estimator/15 -> TraceChannels/15
  Estimator/16 -> TraceChannels/16
  Estimator/17 -> TraceChannels/17
  Estimator/18 -> TraceChannels/18
  Estimator/19 -> TraceChannels/19
  Estimator/20 -> TraceChannels/20
  Estimator/21 -> TraceChannels/21
  Estimator/22 -> TraceChannels/22
  Estimator/23 -> TraceChannels/23
  Estimator/24 -> TraceChannels/24
  Estimator/25 -> TraceChannels/25
  EstimateAngleScopeChannels/1 -> EstimateAngleScope/1
  EstimateSpeedScopeChannels/1 -> EstimateSpeedScope/1
  ResidualScopeChannels/1 -> ResidualScope/1
  ValidityScopeChannels/1 -> ValidityScope/1
  TerminalVoltageScopeChannels/1 -> TerminalVoltageScope/1
  NISScopeChannels/1 -> NISScope/1
  AngleUncertaintyScopeChannels/1 -> AngleUncertaintyScope/1
  SpeedUncertaintyScopeChannels/1 -> SpeedUncertaintyScope/1

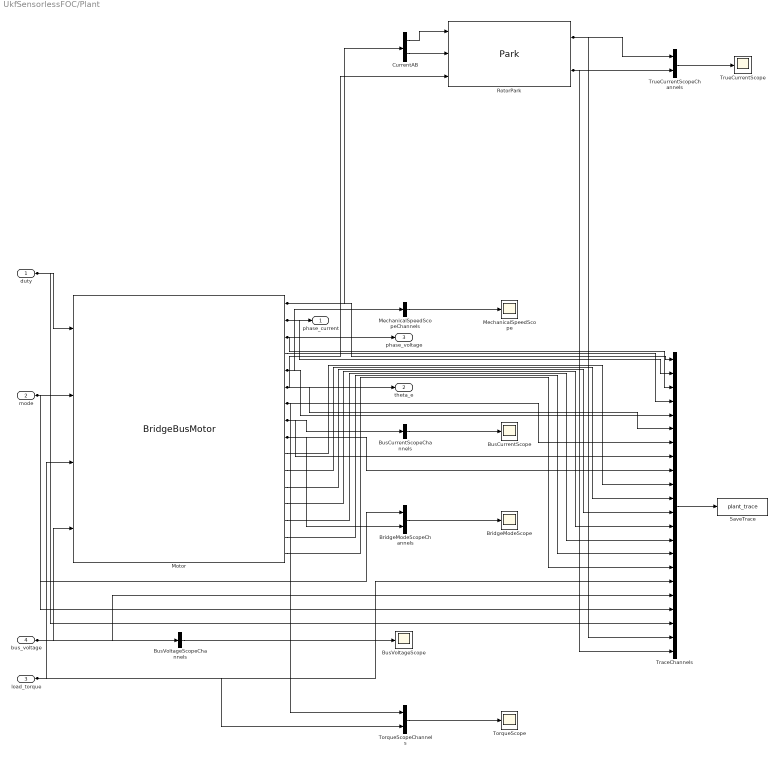
== system UkfSensorlessFOC/Plant ==
  duty : Inport
  mode : Inport  Port=2
  load_torque : Inport  Port=3
  bus_voltage : Inport  Port=4
  BridgeModeScope : Scope
  BridgeModeScopeChannels : Mux  Inputs=2
  BusCurrentScope : Scope
  BusCurrentScopeChannels : Mux  Inputs=1
  BusVoltageScope : Scope
  BusVoltageScopeChannels : Mux  Inputs=1
  CurrentAB : Demux  Outputs=2
  MechanicalSpeedScope : Scope
  MechanicalSpeedScopeChannels : Mux  Inputs=1
  Motor : PMSMBridgeBusPlant/BridgeBusMotor  cfg=bridgeCfg
  RotorPark : ClarkePark/Park  SystemSampleTime=-1  VariantActivationTime=update diagram  EmptyChoice=off  PassThrough=off  PassThroughVariantControl=(default)  EmptyChoiceVariantControl=(default)  AllowFlexibleInterface=on  Latency=0  AutoFrameSizeCalculation=off
  SaveTrace : ToWorkspace  VariableName=plant_trace  SaveFormat=Structure With Time  SampleTime=bridgeCfg.Ts
  TorqueScope : Scope
  TorqueScopeChannels : Mux  Inputs=2
  TraceChannels : Mux  Inputs=22
  TrueCurrentScope : Scope
  TrueCurrentScopeChannels : Mux  Inputs=2
  phase_current : Outport
  theta_e : Outport  Port=2
  phase_voltage : Outport  Port=3
  wires:
  duty/1 -> TraceChannels/20, Motor/1
  mode/1 -> TraceChannels/19, Motor/2, BridgeModeScopeChannels/1
  load_torque/1 -> Motor/3, TraceChannels/17, TorqueScopeChannels/2
  bus_voltage/1 -> BusVoltageScopeChannels/1, Motor/4, TraceChannels/18
  Motor/2 -> TraceChannels/2, phase_current/1
  Motor/6 -> TraceChannels/6, RotorPark/3, theta_e/1
  Motor/3 -> TraceChannels/3, phase_voltage/1
  Motor/1 -> TraceChannels/1, CurrentAB/1
  CurrentAB/1 -> RotorPark/1
  CurrentAB/2 -> RotorPark/2
  TraceChannels/1 -> SaveTrace/1
  Motor/4 -> TraceChannels/4
  Motor/5 -> MechanicalSpeedScopeChannels/1, TraceChannels/5
  Motor/7 -> TorqueScopeChannels/1, TraceChannels/7
  Motor/8 -> BusCurrentScopeChannels/1, TraceChannels/8
  Motor/9 -> BridgeModeScopeChannels/2, TraceChannels/9
  Motor/10 -> TraceChannels/10
  Motor/11 -> TraceChannels/11
  Motor/12 -> TraceChannels/12
  Motor/13 -> TraceChannels/13
  Motor/14 -> TraceChannels/14
  Motor/15 -> TraceChannels/15
  Motor/16 -> TraceChannels/16
  RotorPark/1 -> TrueCurrentScopeChannels/1, TraceChannels/21
  RotorPark/2 -> TrueCurrentScopeChannels/2, TraceChannels/22
  TrueCurrentScopeChannels/1 -> TrueCurrentScope/1
  MechanicalSpeedScopeChannels/1 -> MechanicalSpeedScope/1
  TorqueScopeChannels/1 -> TorqueScope/1
  BusVoltageScopeChannels/1 -> BusVoltageScope/1
  BusCurrentScopeChannels/1 -> BusCurrentScope/1
  BridgeModeScopeChannels/1 -> BridgeModeScope/1

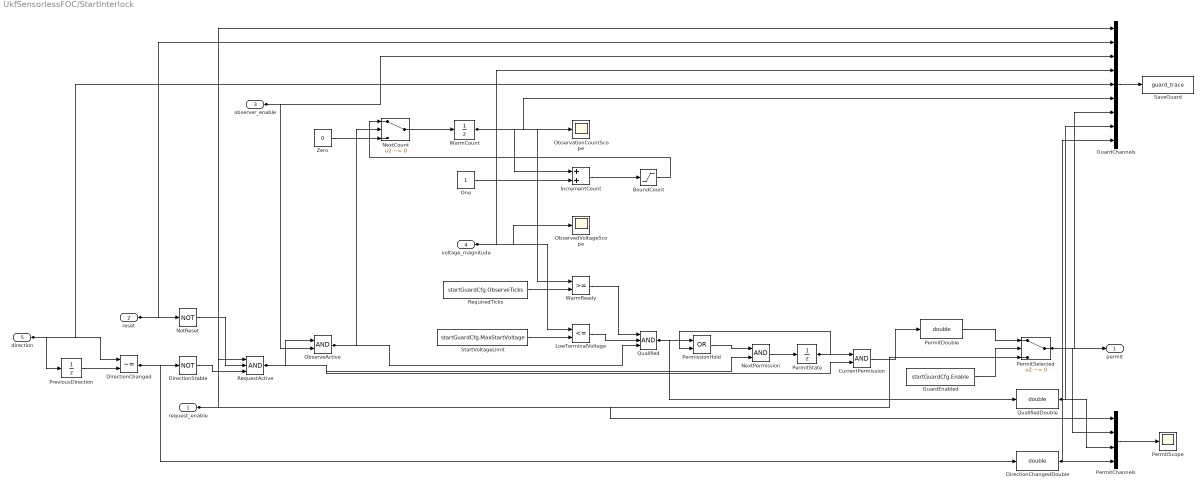
== system UkfSensorlessFOC/StartInterlock ==
  request_enable : Inport
  reset : Inport  Port=2
  observer_enable : Inport  Port=3
  voltage_magnitude : Inport  Port=4
  direction : Inport  Port=5
  BoundCount : Saturate  UpperLimit=startGuardCfg.ObserveTicks  LowerLimit=0
  CurrentPermission : Logic  IconShape=distinctive  AllPortsSameDT=off  OutDataTypeStr=boolean
  DirectionChanged : RelationalOperator  Operator=~=  OutDataTypeStr=boolean  RndMeth=Simplest  InputSameDT=off
  DirectionChangedDouble : DataTypeConversion  OutDataTypeStr=double  SaturateOnIntegerOverflow=off  RndMeth=Floor
  DirectionStable : Logic  Operator=NOT  IconShape=distinctive  AllPortsSameDT=off  OutDataTypeStr=boolean
  GuardChannels : Mux  Inputs=9
  GuardEnabled : Constant  Value=startGuardCfg.Enable
  IncrementCount : Sum
  LowTerminalVoltage : RelationalOperator  Operator=<=  OutDataTypeStr=boolean  RndMeth=Simplest  InputSameDT=off
  NextCount : Switch  Criteria=u2 ~= 0  SaturateOnIntegerOverflow=off  InputSameDT=off
  NextPermission : Logic  IconShape=distinctive  AllPortsSameDT=off  OutDataTypeStr=boolean
  NotReset : Logic  Operator=NOT  IconShape=distinctive  AllPortsSameDT=off  OutDataTypeStr=boolean
  ObservationCountScope : Scope
  ObserveActive : Logic  IconShape=distinctive  AllPortsSameDT=off  OutDataTypeStr=boolean
  ObservedVoltageScope : Scope
  One : Constant
  PermissionHold : Logic  Operator=OR  IconShape=distinctive  AllPortsSameDT=off  OutDataTypeStr=boolean
  PermitChannels : Mux
  PermitDouble : DataTypeConversion  OutDataTypeStr=double  SaturateOnIntegerOverflow=off  RndMeth=Floor
  PermitScope : Scope
  PermitSelected : Switch  Criteria=u2 ~= 0  SaturateOnIntegerOverflow=off  InputSameDT=off
  PermitState : UnitDelay  InitialCondition=false  SampleTime=currentCfg.Ts
  PreviousDirection : UnitDelay  InitialCondition=focCfg.Direction  SampleTime=currentCfg.Ts
  Qualified : Logic  Inputs=3  IconShape=distinctive  AllPortsSameDT=off  OutDataTypeStr=boolean
  QualifiedDouble : DataTypeConversion  OutDataTypeStr=double  SaturateOnIntegerOverflow=off  RndMeth=Floor
  RequestActive : Logic  Inputs=3  IconShape=distinctive  AllPortsSameDT=off  OutDataTypeStr=boolean
  RequiredTicks : Constant  Value=startGuardCfg.ObserveTicks
  SaveGuard : ToWorkspace  VariableName=guard_trace  SaveFormat=Structure With Time  SampleTime=currentCfg.Ts
  StartVoltageLimit : Constant  Value=startGuardCfg.MaxStartVoltage
  WarmCount : UnitDelay  SampleTime=currentCfg.Ts
  WarmReady : RelationalOperator  OutDataTypeStr=boolean  RndMeth=Simplest  InputSameDT=off
  Zero : Constant  Value=0
  permit : Outport
  wires:
  DirectionChangedDouble/1 -> GuardChannels/9, PermitChannels/4
  QualifiedDouble/1 -> GuardChannels/8, PermitChannels/3
  PermitChannels/1 -> PermitScope/1
  GuardChannels/1 -> SaveGuard/1
  PermitSelected/1 -> permit/1, GuardChannels/7, PermitChannels/2
  GuardEnabled/1 -> PermitSelected/2
  PermitDouble/1 -> PermitSelected/1
  CurrentPermission/1 -> PermitDouble/1
  NextPermission/1 -> PermitState/1
  PermissionHold/1 -> NextPermission/1
  PermitState/1 -> PermissionHold/2, CurrentPermission/1
  Qualified/1 -> PermissionHold/1, QualifiedDouble/1
  LowTerminalVoltage/1 -> Qualified/2
  WarmReady/1 -> Qualified/1
  StartVoltageLimit/1 -> LowTerminalVoltage/2
  voltage_magnitude/1 -> LowTerminalVoltage/1, ObservedVoltageScope/1, GuardChannels/4
  RequiredTicks/1 -> WarmReady/2
  NextCount/1 -> WarmCount/1
  Zero/1 -> NextCount/3
  ObserveActive/1 -> NextCount/2, Qualified/3
  BoundCount/1 -> NextCount/1
  IncrementCount/1 -> BoundCount/1
  One/1 -> IncrementCount/2
  WarmCount/1 -> WarmReady/1, IncrementCount/1, ObservationCountScope/1, GuardChannels/6
  observer_enable/1 -> ObserveActive/2, GuardChannels/3
  RequestActive/1 -> ObserveActive/1, NextPermission/2, CurrentPermission/2
  DirectionStable/1 -> RequestActive/3
  NotReset/1 -> RequestActive/2
  request_enable/1 -> RequestActive/1, PermitSelected/3, GuardChannels/1, PermitChannels/1
  reset/1 -> NotReset/1, GuardChannels/2
  DirectionChanged/1 -> DirectionChangedDouble/1, DirectionStable/1
  PreviousDirection/1 -> DirectionChanged/2
  direction/1 -> PreviousDirection/1, DirectionChanged/1, GuardChannels/5

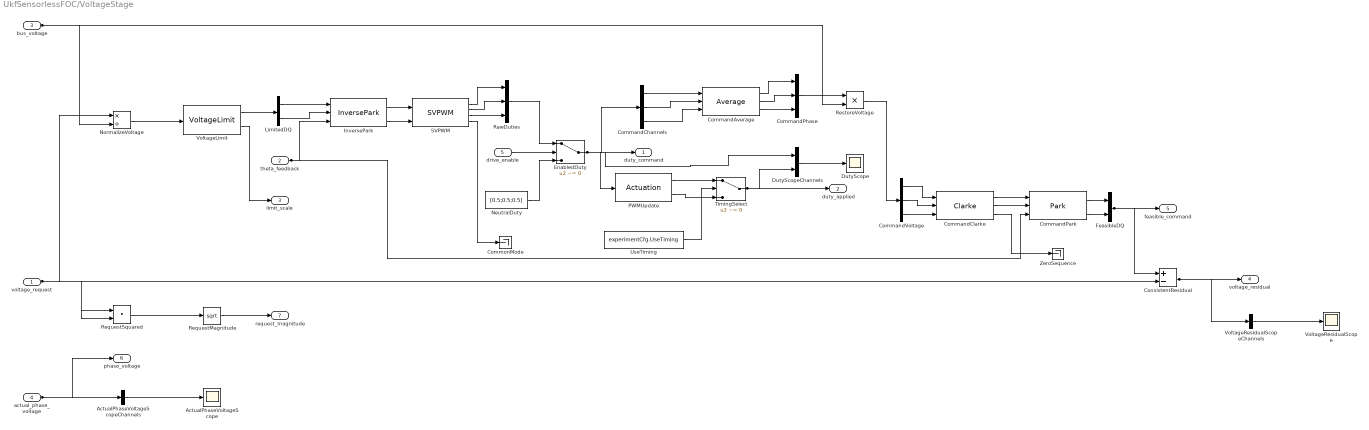
== system UkfSensorlessFOC/VoltageStage ==
  voltage_request : Inport
  theta_feedback : Inport  Port=2
  bus_voltage : Inport  Port=3
  actual_phase_voltage : Inport  Port=4
  drive_enable : Inport  Port=5
  ActualPhaseVoltageScope : Scope
  ActualPhaseVoltageScopeChannels : Mux  Inputs=1
  CommandAverage : Inverter/Average  SystemSampleTime=-1  VariantActivationTime=update diagram  EmptyChoice=off  PassThrough=off  PassThroughVariantControl=(default)  EmptyChoiceVariantControl=(default)  AllowFlexibleInterface=on  Latency=0  AutoFrameSizeCalculation=off
  CommandChannels : Demux  Outputs=3
  CommandClarke : ClarkePark/Clarke  SystemSampleTime=-1  VariantActivationTime=update diagram  EmptyChoice=off  PassThrough=off  PassThroughVariantControl=(default)  EmptyChoiceVariantControl=(default)  AllowFlexibleInterface=on  Latency=0  AutoFrameSizeCalculation=off
  CommandPark : ClarkePark/Park  SystemSampleTime=-1  VariantActivationTime=update diagram  EmptyChoice=off  PassThrough=off  PassThroughVariantControl=(default)  EmptyChoiceVariantControl=(default)  AllowFlexibleInterface=on  Latency=0  AutoFrameSizeCalculation=off
  CommandPhase : Mux  Inputs=3
  CommandVoltage : Demux  Outputs=3
  CommonMode : Terminator
  ConsistentResidual : Sum  Inputs=+-
  DutyScope : Scope
  DutyScopeChannels : Mux  Inputs=2
  EnabledDuty : Switch  Criteria=u2 ~= 0  SaturateOnIntegerOverflow=off  InputSameDT=off
  FeasibleDQ : Mux  Inputs=2
  InversePark : ClarkePark/InversePark  SystemSampleTime=-1  VariantActivationTime=update diagram  EmptyChoice=off  PassThrough=off  PassThroughVariantControl=(default)  EmptyChoiceVariantControl=(default)  AllowFlexibleInterface=on  Latency=0  AutoFrameSizeCalculation=off
  LimitedDQ : Demux  Outputs=2
  NeutralDuty : Constant  Value=[0.5;0.5;0.5]
  NormalizeVoltage : Product  Inputs=*/
  PWMUpdate : ControlTiming/Actuation  SystemSampleTime=-1  VariantActivationTime=update diagram  EmptyChoice=off  PassThrough=off  PassThroughVariantControl=(default)  EmptyChoiceVariantControl=(default)  AllowFlexibleInterface=on  Latency=0  AutoFrameSizeCalculation=off
  RawDuties : Mux  Inputs=3
  RequestMagnitude : Sqrt
  RequestSquared : DotProduct  OutDataTypeStr=Inherit: Inherit via internal rule
  RestoreVoltage : Product  Inputs=**
  SVPWM : Inverter/SVPWM  SystemSampleTime=-1  VariantActivationTime=update diagram  EmptyChoice=off  PassThrough=off  PassThroughVariantControl=(default)  EmptyChoiceVariantControl=(default)  AllowFlexibleInterface=on  Latency=0  AutoFrameSizeCalculation=off
  TimingSelect : Switch  Criteria=u2 ~= 0  SaturateOnIntegerOverflow=off  InputSameDT=off
  UseTiming : Constant  Value=experimentCfg.UseTiming
  VoltageLimit : CurrentControl/VoltageLimit  SystemSampleTime=-1  VariantActivationTime=update diagram  EmptyChoice=off  PassThrough=off  PassThroughVariantControl=(default)  EmptyChoiceVariantControl=(default)  AllowFlexibleInterface=on  Latency=0  AutoFrameSizeCalculation=off
  VoltageResidualScope : Scope
  VoltageResidualScopeChannels : Mux  Inputs=1
  ZeroSequence : Terminator
  duty_command : Outport
  duty_applied : Outport  Port=2
  limit_scale : Outport  Port=3
  voltage_residual : Outport  Port=4
  feasible_command : Outport  Port=5
  phase_voltage : Outport  Port=6
  request_magnitude : Outport  Port=7
  wires:
  voltage_request/1 -> RequestSquared/2, RequestSquared/1, NormalizeVoltage/1, ConsistentResidual/2
  bus_voltage/1 -> RestoreVoltage/2, NormalizeVoltage/2
  NormalizeVoltage/1 -> VoltageLimit/1
  VoltageLimit/1 -> LimitedDQ/1
  LimitedDQ/1 -> InversePark/1
  LimitedDQ/2 -> InversePark/2
  theta_feedback/1 -> CommandPark/3, InversePark/3
  InversePark/1 -> SVPWM/1
  InversePark/2 -> SVPWM/2
  SVPWM/4 -> CommonMode/1
  RawDuties/1 -> EnabledDuty/1
  drive_enable/1 -> EnabledDuty/2
  NeutralDuty/1 -> EnabledDuty/3
  EnabledDuty/1 -> duty_command/1, PWMUpdate/1, DutyScopeChannels/1, CommandChannels/1
  PWMUpdate/1 -> TimingSelect/1
  UseTiming/1 -> TimingSelect/2
  PWMUpdate/2 -> TimingSelect/3
  TimingSelect/1 -> DutyScopeChannels/2, duty_applied/1
  CommandPhase/1 -> RestoreVoltage/1
  RestoreVoltage/1 -> CommandVoltage/1
  CommandClarke/1 -> CommandPark/1
  CommandClarke/2 -> CommandPark/2
  CommandClarke/3 -> ZeroSequence/1
  CommandPark/1 -> FeasibleDQ/1
  CommandPark/2 -> FeasibleDQ/2
  FeasibleDQ/1 -> ConsistentResidual/1, feasible_command/1
  ConsistentResidual/1 -> VoltageResidualScopeChannels/1, voltage_residual/1
  VoltageLimit/2 -> limit_scale/1
  actual_phase_voltage/1 -> ActualPhaseVoltageScopeChannels/1, phase_voltage/1
  RequestSquared/1 -> RequestMagnitude/1
  RequestMagnitude/1 -> request_magnitude/1
  SVPWM/1 -> RawDuties/1
  CommandChannels/1 -> CommandAverage/1
  CommandAverage/1 -> CommandPhase/1
  CommandVoltage/1 -> CommandClarke/1
  SVPWM/2 -> RawDuties/2
  CommandChannels/2 -> CommandAverage/2
  CommandAverage/2 -> CommandPhase/2
  CommandVoltage/2 -> CommandClarke/2
  SVPWM/3 -> RawDuties/3
  CommandChannels/3 -> CommandAverage/3
  CommandAverage/3 -> CommandPhase/3
  CommandVoltage/3 -> CommandClarke/3
  DutyScopeChannels/1 -> DutyScope/1
  VoltageResidualScopeChannels/1 -> VoltageResidualScope/1
  ActualPhaseVoltageScopeChannels/1 -> ActualPhaseVoltageScope/1
